simulink model "mech_state"  (R2023a)
settings: Solver=ode45  StartTime=0.0  StopTime=5  RelTol=1e-3
settings Model: Creator=ahmad  LastModifiedBy=ahmad

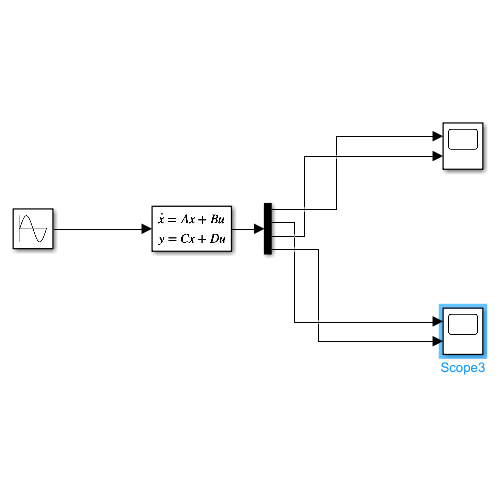
[thumbnail: Simulink's stored preview of the top-level diagram]
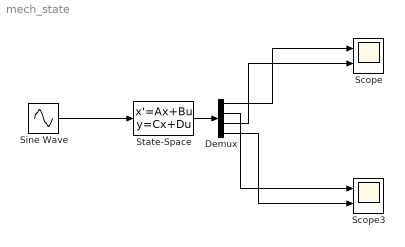
== system mech_state ==
  Demux : Demux
  Scope : Scope  NumInputPorts=2
  Scope3 : Scope  NumInputPorts=2
  Sine Wave : Sin  Amplitude=5000  Frequency=8*pi  SampleTime=0
  State-Space : StateSpace  A=[0, 1, 0, 0; -1050, -1500, 50, 500; 0, 0, 0, 1; 1000, 10000, -1000, -10000]  B=[0; 0.00025; 0; 0]  C=[1, 0, 0, 0; 0, 1, 0, 0; 0, 0, 1, 0; 0, 0, 0, 1]  D=[0; 0; 0; 0]  InitialCondition=[0 0 0 0]
  wires:
  Sine Wave/1 -> State-Space/1
  State-Space/1 -> Demux/1
  Demux/1 -> Scope/1
  Demux/2 -> Scope3/1
  Demux/4 -> Scope3/2
  Demux/3 -> Scope/2
